simulink model "HW1_7_DOB_r1_yes"  (R2025a)
settings: Solver=VariableStepAuto  StartTime=0.0  StopTime=5  RelTol=1e-3
settings Model: Creator=BCC  LastModifiedBy=BCC

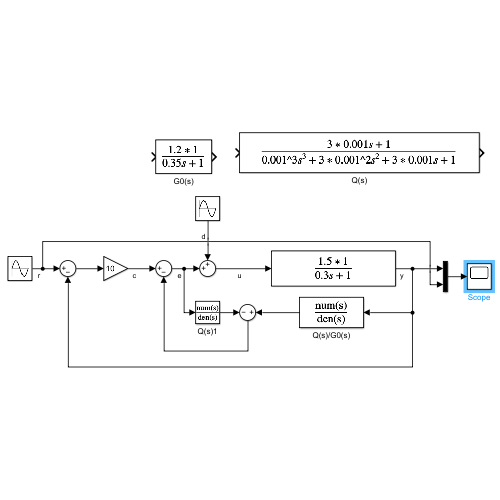
[thumbnail: Simulink's stored preview of the top-level diagram]
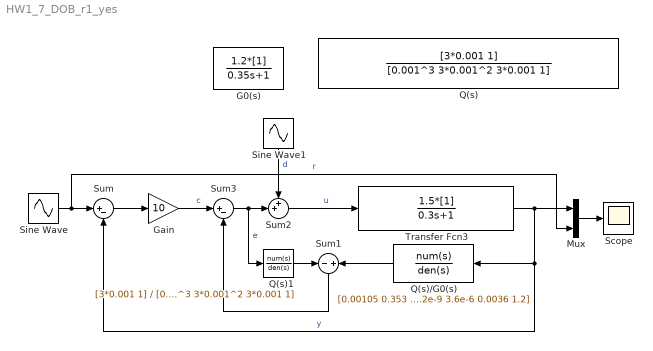
== system HW1_7_DOB_r1_yes ==
  G0(s) : TransferFcn  Numerator=1.2*[1]  Denominator=[0.35 1]
  Gain : Gain  Gain=10
  Mux : Mux  Inputs=2
  Q(s) : TransferFcn  Numerator=[3*0.001 1]  Denominator=[0.001^3 3*0.001^2 3*0.001 1]
  Q(s)/G0(s) : TransferFcn  Numerator=[0.00105 0.353 1]  Denominator=[1.2e-9 3.6e-6 0.0036 1.2]
  Q(s)1 : TransferFcn  Numerator=[3*0.001 1]  Denominator=[0.001^3 3*0.001^2 3*0.001 1]
  Scope : Scope
      settings: ActiveDisplayYMinimum=-1.7538217253697685  ActiveDisplayYMaximum=1.751561250264799
  Sine Wave : Sin  Frequency=2*pi*2  SampleTime=0
  Sine Wave1 : Sin  Amplitude=5  Frequency=2*pi*200  SampleTime=0
  Sum : Sum  Inputs=|+-
  Sum1 : Sum  Inputs=-+
  Sum2 : Sum  Inputs=++|  CollapseMode=Specified dimension  CollapseDim=2
  Sum3 : Sum  Inputs=|+-
  Transfer Fcn3 : TransferFcn  Numerator=1.5*[1]  Denominator=[0.3 1]
  wires:
  Sine Wave/1 -> Mux/2, Sum/1  "r"
  Sum/1 -> Gain/1
  Transfer Fcn3/1 -> Mux/1, Sum/2, Q(s)/G0(s)/1  "y"
  Sine Wave1/1 -> Sum2/1  "d"
  Sum2/1 -> Transfer Fcn3/1  "u"
  Mux/1 -> Scope/1
  Gain/1 -> Sum3/1  "c"
  Sum3/1 -> Q(s)1/1, Sum2/2  "e"
  Q(s)/G0(s)/1 -> Sum1/2
  Q(s)1/1 -> Sum1/1
  Sum1/1 -> Sum3/2
